simulink model "buffer_test"  (R2025b)
settings: Solver=VariableStepAuto  StartTime=0.0  StopTime=10.0  RelTol=1e-3
libraries: dspxfrm3 x1
settings Model: Creator=Yahin  LastModifiedBy=Yahin

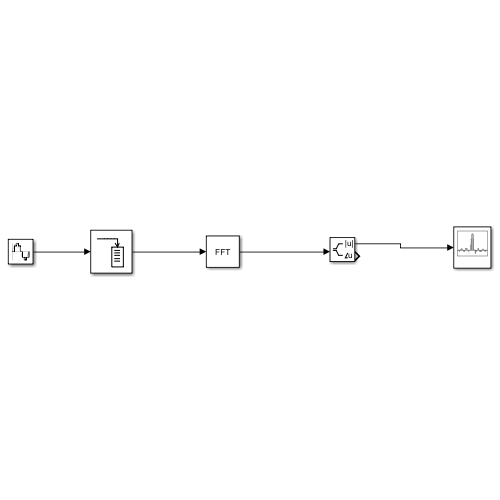
[thumbnail: Simulink's stored preview of the top-level diagram]
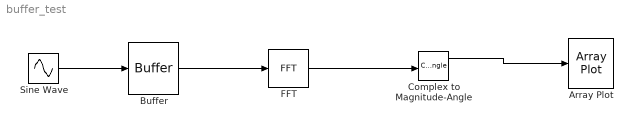
== system buffer_test ==
  Array Plot : ArrayPlot  WindowPosition=[560.000000,290.000000,800.000000,500.000000,]  ScopeFrameLocation=window  YLimits=[-47.8071 436.1414]
  Buffer : Buffer  N=1024  OutputFrames=off
  Complex to Magnitude-Angle : ComplexToMagnitudeAngle
  FFT : dspxfrm3/FFT  FFTImplementation=Auto  CompMethod=Table lookup  TableOpt=NEW  TableOptActive=Speed  BitRevOrder=off  Normalize=off  InheritFFTLength=on  FFTLength=64  WrapInput=on  roundingMode=Ceiling  overflowMode=off  firstCoeffDataTypeStr=Inherit: Same word length as input  firstCoeffLastDataTypeStr=Inherit: Same word length as input  outputMin=[]  outputMax=[]
  Sine Wave : Sin  Frequency=2*pi*100  SampleTime=1/1000
  wires:
  FFT/1 -> Complex to Magnitude-Angle/1
  Sine Wave/1 -> Buffer/1
  Complex to Magnitude-Angle/1 -> Array Plot/1
  Buffer/1 -> FFT/1
